simulink library "tip_assist_lib_support"  (Simulink 9.0)
settings: Solver=VariableStepAuto  StartTime=0.0  StopTime=10.0  RelTol=1e-3
undefined symbols (not defined in the file): g, timestep, TipAssistAdvEcmError_t, TipAssistCpmTipOffMode_t, TipAssistLiveWeighStatus_t, TipAssistPayloadType_t, TipAssistSecPfwStatus_t, TipAssistUnsecPfwStatus_t, toa_appNumber, toa_expectedBucketAngNoise, toa_imu_lpf_cutoff_hz, toa_imuBasicOrient, toa_liftBoreDia, toa_liftRodDia, toa_liveLpfCutoffHz, toa_liveSpillRateLpfCutoffHz, toa_mcGroundCombBucketAng, toa_mcGroundCombLiftNormAng, toa_mcGroundLiftNormAng, toa_noSlidingAngle, toa_payload_target_ov_val, toa_payloadTargetMin, toa_pfwLpfCutoffHz, toa_pfwResetLpfCutoffHz, toa_pfwResetStatsBound, toa_pfwResetStatsConf, toa_pfwTiltNormRackThresh, toa_pfwTravelExtentLower, toa_pfwTravelExtentUpper, toa_ratedPayload, toa_reposeMarginAng, toa_sendCpmLiveLpfCutoffHz, toa_sendToCpmMinPrecision, toa_tiltBoreDia, toa_tiltNumCyl, toa_tiltRodDia, toa_toolBcAngle, toa_toolBcLength
libraries: lib_CATutils_Utilities_ApplyName_v2 x113, simulink x18, tip_assist_lib x14, lib_CATutils_Filters_1Pole_LowPass x6, simulink_extras x5, lib_CATutils_Override x3, lib_CATutils_Hysteresis_Latch x3, lib_CATutils_Timer_Countdown x3, tip_assist_lib_support x2
(part 4 of 4)

== matlab function Tip-Off Assist Support Lib/Tip-Off Assist Payload/Pseudo-Frictionless Weigh/Weighing Statistics, Notch, No Latch/Two Sided Confidence Limit ==
  data: confidence input double; bound output double; stdev input double
function bound = TwoSidedConfBound(confidence, stdev)
% Calculates the size of a confidence interval in terms of half its width.
%
% Inputs:
%   confidence
%   Confidence that the resulting bound will enclose the true value.
%
%   stdev
%   The observed standard deviation, expressed in the same units as
%   bound. Can be thought of as defining the scale of the normal
%   distribution that we are assuming represents the data we are sampling.
%
%   Potential units for the arguments are percent of rated payload or
%   payload.
%
% Outputs:
%   bound
%   Bound of the confidence interval, expressed in the same units as stdev.
%   
%   For lower bound, the true value will lie above the mean minus this
%   value.
%   The opposite is true for an upper bound.
%   
% Inspired from pcs_calculate_confidence() in pcs_io.c

% Table of confidence vs two-sided confidence interval bound.
% Units of confidence decimal percent and the ratio of standard
% deviation of a standard normal distribution.
xConfidenceTwoSided = [ 0.0, 0.235822844, 0.382924922, 0.516072694, 0.631879747, 0.728667676, 0.806398927, 0.866385543, 0.910869057, 0.942566872, 0.964271153, 0.978551778, 0.987580668, 0.993066052, 0.997300204, 0.999534742, 1.0 ];
yStdevRatio = [ 0.0, 0.3, 0.5, 0.7, 0.9, 1.1, 1.3, 1.5, 1.7, 1.9, 2.1, 2.3, 2.5, 2.7, 3.0, 3.5, 4.0 ];
stdev_ratio = interp1(xConfidenceTwoSided, yStdevRatio, confidence);
bound = stdev_ratio * stdev;

== matlab function Tip-Off Assist Support Lib/EEF IMU to NEEF gravity vector/EEF vector to NEEF vector ==
  data: eefVector input double; neefVector output double; steeringAngle input double
function neefVector  = fcn(eefVector, steeringAngle)
% Transforms a vector on the EEF to a vector on the NEEF via steering angle
rotAxis = [0; 1; 0];               % Steering right is positive angle
angle = steeringAngle;

% Form rotation matrix
crossProductMatrix = [
    0,          -rotAxis(3),  rotAxis(2);
     rotAxis(3), 0,          -rotAxis(1);
    -rotAxis(2), rotAxis(1),  0
];
tensorProduct = rotAxis * transpose(rotAxis);
rotMatrix = cos(angle) * eye(3) + sin(angle) * crossProductMatrix + ...
    (1 - cos(angle)) * tensorProduct;

neefVector = rotMatrix * eefVector;

== matlab function Tip-Off Assist Support Lib/Tip-Off Assist Payload/Pseudo-Frictionless Weigh/Weighing Statistics, Notch, No Latch/One Sided Confidence Limit ==
  data: confidence input double; bound output double; stdev input double
function bound = oneSidedConfBound(confidence, stdev)
% Calculates the size of a confidence interval in terms of half its width.
%
% Inputs:
%   confidence
%   Confidence that the resulting bound will enclose the true value.
%
%   stdev
%   The observed standard deviation, expressed in the same units as
%   bound. Can be thought of as defining the scale of the normal
%   distribution that we are assuming represents the data we are sampling.
%
%   Potential units for the arguments are percent of rated payload or
%   payload.
%
% Outputs:
%   bound
%   Bound of the confidence interval, expressed in the same units as stdev.
%   
%   For lower bound, the true value will lie above the mean minus this
%   value.
%   The opposite is true for an upper bound.
%   
% Inspired from pcs_calculate_confidence() in pcs_io.c

% Table of confidence vs one-sided confidence interval bound.
% Units of confidence decimal percent and the ratio of standard
% deviation of a standard normal distribution.
xConfidenceOneSided = [0.500000000000000,0.617911422000000,0.691462461000000,0.758036347000000,0.815939873500000,0.864333838000000,0.903199463500000,0.933192771500000,0.955434528500000,0.971283436000000,0.982135576500000,0.989275889000000,0.993790334000000,0.996533026000000,0.998650102000000,0.999767371000000,1];
yStdevRatio = [ 0.0, 0.3, 0.5, 0.7, 0.9, 1.1, 1.3, 1.5, 1.7, 1.9, 2.1, 2.3, 2.5, 2.7, 3.0, 3.5, 4.0 ];
stdev_ratio = interp1(xConfidenceOneSided, yStdevRatio, confidence);
bound = stdev_ratio * stdev;

== matlab function Tip-Off Assist Support Lib/EEF IMU to NEEF gravity vector/euler angles from rot matrix ==
  data: rotations output double; rotMatrix input double
function rotations  = decomp(rotMatrix)
%   Input:  3x3 rotation matrix
%   Output: 1x3 vector of euler angles in degrees
rotations = zeros(1,3);
rotations(1) = atan2(rotMatrix(3,2),rotMatrix(3,3));
rotations(2) = atan2(-rotMatrix(3,1), (sqrt((rotMatrix(3,2)^2)+(rotMatrix(3,3)^2))));
rotations(3) = atan2(rotMatrix(2,1),rotMatrix(1,1));
% convert back to degrees
for i=1:size(rotations,2)
    rotations(i) = 180*rotations(i)/pi;
end
end

== matlab function Tip-Off Assist Support Lib/Tip-Off Assist Payload/Pseudo-Frictionless Weigh/Weighing Statistics, No Notch, No Latch/One Sided Confidence Limit ==
  data: confidence input double; bound output double; stdev input double
function bound = oneSidedConfBound(confidence, stdev)
% Calculates the size of a confidence interval in terms of half its width.
%
% Inputs:
%   confidence
%   Confidence that the resulting bound will enclose the true value.
%
%   stdev
%   The observed standard deviation, expressed in the same units as
%   bound. Can be thought of as defining the scale of the normal
%   distribution that we are assuming represents the data we are sampling.
%
%   Potential units for the arguments are percent of rated payload or
%   payload.
%
% Outputs:
%   bound
%   Bound of the confidence interval, expressed in the same units as stdev.
%   
%   For lower bound, the true value will lie above the mean minus this
%   value.
%   The opposite is true for an upper bound.
%   
% Inspired from pcs_calculate_confidence() in pcs_io.c

% Table of confidence vs one-sided confidence interval bound.
% Units of confidence decimal percent and the ratio of standard
% deviation of a standard normal distribution.
xConfidenceOneSided = [0.500000000000000,0.617911422000000,0.691462461000000,0.758036347000000,0.815939873500000,0.864333838000000,0.903199463500000,0.933192771500000,0.955434528500000,0.971283436000000,0.982135576500000,0.989275889000000,0.993790334000000,0.996533026000000,0.998650102000000,0.999767371000000,1];
yStdevRatio = [ 0.0, 0.3, 0.5, 0.7, 0.9, 1.1, 1.3, 1.5, 1.7, 1.9, 2.1, 2.3, 2.5, 2.7, 3.0, 3.5, 4.0 ];
stdev_ratio = interp1(xConfidenceOneSided, yStdevRatio, confidence);
bound = stdev_ratio * stdev;

== matlab function Tip-Off Assist Support Lib/Tip-Off Assist Payload/Pseudo-Frictionless Weigh/Weighing Statistics, No Notch, No Latch/Two Sided Confidence Limit ==
  data: confidence input double; bound output double; stdev input double
function bound = TwoSidedConfBound(confidence, stdev)
% Calculates the size of a confidence interval in terms of half its width.
%
% Inputs:
%   confidence
%   Confidence that the resulting bound will enclose the true value.
%
%   stdev
%   The observed standard deviation, expressed in the same units as
%   bound. Can be thought of as defining the scale of the normal
%   distribution that we are assuming represents the data we are sampling.
%
%   Potential units for the arguments are percent of rated payload or
%   payload.
%
% Outputs:
%   bound
%   Bound of the confidence interval, expressed in the same units as stdev.
%   
%   For lower bound, the true value will lie above the mean minus this
%   value.
%   The opposite is true for an upper bound.
%   
% Inspired from pcs_calculate_confidence() in pcs_io.c

% Table of confidence vs two-sided confidence interval bound.
% Units of confidence decimal percent and the ratio of standard
% deviation of a standard normal distribution.
xConfidenceTwoSided = [ 0.0, 0.235822844, 0.382924922, 0.516072694, 0.631879747, 0.728667676, 0.806398927, 0.866385543, 0.910869057, 0.942566872, 0.964271153, 0.978551778, 0.987580668, 0.993066052, 0.997300204, 0.999534742, 1.0 ];
yStdevRatio = [ 0.0, 0.3, 0.5, 0.7, 0.9, 1.1, 1.3, 1.5, 1.7, 1.9, 2.1, 2.3, 2.5, 2.7, 3.0, 3.5, 4.0 ];
stdev_ratio = interp1(xConfidenceTwoSided, yStdevRatio, confidence);
bound = stdev_ratio * stdev;

== matlab function Tip-Off Assist Support Lib/EEF IMU to NEEF gravity vector/rotation matrix calc from two vectors ==
  data: level_vec_meas input double; rotMatrix output double; level_vec_act input double; rotAxis output double; angle output double
function [rotMatrix, rotAxis, angle] = fcn(level_vec_meas, level_vec_act)
% Should match output of:
%     vrrotvec2mat(vrrotvec(level_vec_meas, level_vec_act))

if all(level_vec_meas == level_vec_act)
    % No transform necessary, return identity matrix
    rotAxis = single([9999; 9999; 9999]);
    angle = single(9999);
    rotMatrix = single(eye(3));
    return
end
    
a = level_vec_meas;
b = level_vec_act;

cp = cross(a, b);
cpNorm = norm(cp);

rotAxis = cp/cpNorm;
angle_rad = atan(cpNorm/dot(a, b));
angle = angle_rad * 180.0 / pi;

% Form rotation matrix
crossProductMatrix = [
    0,          -rotAxis(3),  rotAxis(2);
     rotAxis(3), 0,          -rotAxis(1);
    -rotAxis(2), rotAxis(1),  0
];
tensorProduct = rotAxis * transpose(rotAxis);
rotMatrix = cos(angle_rad) * eye(3) + sin(angle_rad) * crossProductMatrix + ...
    (1 - cos(angle_rad)) * tensorProduct;

== matlab function Tip-Off Assist Support Lib/Tip-Off Assist Payload/Pseudo-Frictionless Weigh/Variance Anti-Noise Filter1/MATLAB Function ==
  data: u input double; y output double; reset input double
function y = movingAverage(u, reset)

persistent lastSample
if isempty(lastSample) || reset
    lastSample = u;
end
y = (u + lastSample) / 2;
lastSample = u;

== stateflow chart Tip-Off Assist Support Lib/Tip-Off Assist Payload/Pseudo-Frictionless Weigh/Notch filter/NotchFilter/Filter ==
  state Update
    du: updateFilter();
  state initFilter [function]
    (default) -> (junction 133) : {
        | q = (cf*cf*ts*ts)/4.0c;
        | r = cf*ts;
        | p = 1.0c + q;
        | s = 2.0c * (q - 1.0c);
        | t = p + r;
        |
        | alpha = p / t;
        | beta = s / t;
        | gamma = r / t;
        | }
    (junction 133) -> (junction 134) : {
        | rawHist[0] = raw;
        | rawHist[1] = raw;
        | rawHist[2] = raw;
        | }
    (junction 134) -> (junction 135) : {
        | filtHist[0] = raw;
        | filtHist[1] = raw;
        | filtHist[2] = raw;
        | }
    (junction 135) -> (junction 136) : {
        | filtered = filtHist[0];
        | }
  state updateFilter [function]
    (default) -> (junction 141) : {
        | rawHist[2] = rawHist[1];
        | rawHist[1] = rawHist[0];
        | rawHist[0] = raw;
        | }
    (junction 141) -> (junction 142) : {
        | filtHist[2] = filtHist[1];
        | filtHist[1] = filtHist[0];
        | filtHist[0] = (alpha * (rawHist[0] + rawHist[2] - filtHist[2])) + (beta * (rawHist[1] - filtHist[1])) + (gamma * filtHist[2]);
        | }
    (junction 142) -> (junction 143) : {
        | filtered = filtHist[0];
        | }
  (default) -> (junction 157)
  Update -> (junction 157) : [reset]
  (junction 157) -> Update : {initFilter();}
  data: q temporary single; r temporary single; p temporary single; s temporary single; t temporary single; raw input single; reset input boolean; ts input single; cf input single; filtered output single; rawHist local single size=3; filtHist local single size=3; alpha local single; beta local single; gamma local single

== stateflow chart Tip-Off Assist Support Lib/Tip-Off Assist Payload/Pseudo-Frictionless Weigh/Notch filter/NotchFilter1/Filter ==
  state Update
    du: updateFilter();
  state initFilter [function]
    (default) -> (junction 171) : {
        | q = (cf*cf*ts*ts)/4.0c;
        | r = cf*ts;
        | p = 1.0c + q;
        | s = 2.0c * (q - 1.0c);
        | t = p + r;
        |
        | alpha = p / t;
        | beta = s / t;
        | gamma = r / t;
        | }
    (junction 171) -> (junction 172) : {
        | rawHist[0] = raw;
        | rawHist[1] = raw;
        | rawHist[2] = raw;
        | }
    (junction 172) -> (junction 173) : {
        | filtHist[0] = raw;
        | filtHist[1] = raw;
        | filtHist[2] = raw;
        | }
    (junction 173) -> (junction 174) : {
        | filtered = filtHist[0];
        | }
  state updateFilter [function]
    (default) -> (junction 179) : {
        | rawHist[2] = rawHist[1];
        | rawHist[1] = rawHist[0];
        | rawHist[0] = raw;
        | }
    (junction 179) -> (junction 180) : {
        | filtHist[2] = filtHist[1];
        | filtHist[1] = filtHist[0];
        | filtHist[0] = (alpha * (rawHist[0] + rawHist[2] - filtHist[2])) + (beta * (rawHist[1] - filtHist[1])) + (gamma * filtHist[2]);
        | }
    (junction 180) -> (junction 181) : {
        | filtered = filtHist[0];
        | }
  (default) -> (junction 195)
  Update -> (junction 195) : [reset]
  (junction 195) -> Update : {initFilter();}
  data: q temporary single; r temporary single; p temporary single; s temporary single; t temporary single; raw input single; reset input boolean; ts input single; cf input single; filtered output single; rawHist local single size=3; filtHist local single size=3; alpha local single; beta local single; gamma local single

== stateflow chart Tip-Off Assist Support Lib/Tip-Off Assist Payload/Pseudo-Frictionless Weigh/Notch filter/NotchFilter2/Filter ==
  state Update
    du: updateFilter();
  state initFilter [function]
    (default) -> (junction 209) : {
        | q = (cf*cf*ts*ts)/4.0c;
        | r = cf*ts;
        | p = 1.0c + q;
        | s = 2.0c * (q - 1.0c);
        | t = p + r;
        |
        | alpha = p / t;
        | beta = s / t;
        | gamma = r / t;
        | }
    (junction 209) -> (junction 210) : {
        | rawHist[0] = raw;
        | rawHist[1] = raw;
        | rawHist[2] = raw;
        | }
    (junction 210) -> (junction 211) : {
        | filtHist[0] = raw;
        | filtHist[1] = raw;
        | filtHist[2] = raw;
        | }
    (junction 211) -> (junction 212) : {
        | filtered = filtHist[0];
        | }
  state updateFilter [function]
    (default) -> (junction 217) : {
        | rawHist[2] = rawHist[1];
        | rawHist[1] = rawHist[0];
        | rawHist[0] = raw;
        | }
    (junction 217) -> (junction 218) : {
        | filtHist[2] = filtHist[1];
        | filtHist[1] = filtHist[0];
        | filtHist[0] = (alpha * (rawHist[0] + rawHist[2] - filtHist[2])) + (beta * (rawHist[1] - filtHist[1])) + (gamma * filtHist[2]);
        | }
    (junction 218) -> (junction 219) : {
        | filtered = filtHist[0];
        | }
  (default) -> (junction 233)
  Update -> (junction 233) : [reset]
  (junction 233) -> Update : {initFilter();}
  data: q temporary single; r temporary single; p temporary single; s temporary single; t temporary single; raw input single; reset input boolean; ts input single; cf input single; filtered output single; rawHist local single size=3; filtHist local single size=3; alpha local single; beta local single; gamma local single

== matlab function Tip-Off Assist Support Lib/Tip-Off Assist Payload/Pseudo-Frictionless Weigh/Statistics Estimation1/Two Sided St. Dev. from Bound ==
  data: confidence input double; stdev output double; bound input double
function stdev = TwoSidedConfBound(confidence, bound)
% Calculates the st. dev. of a confidence interval in terms of half its width.
%
% Inputs:
%   confidence
%   Confidence that the input bound will enclose the true value.
%
%   bound
%   Bound of the confidence interval, expressed in the same units as stdev.
%   
%   For lower bound, the true value will lie above the mean minus this
%   value.
%   The opposite is true for an upper bound.
%
%   Potential units for the arguments are percent of rated payload or
%   payload.
%
% Outputs:
%   stdev
%   The standard deviation, expressed in the same units as
%   bound, that corresponds to the given bound. Can be thought of as
%   describing the scale of the normal distribution whose confidence
%   interval with given bounds results in the given confidence.
%   
% Inspired from pcs_calculate_confidence() in pcs_io.c

% Table of confidence vs two-sided confidence interval bound.
% Units of confidence decimal percent and the ratio of standard
% deviation of a standard normal distribution.
xConfidenceTwoSided = [ 0.0, 0.235822844, 0.382924922, 0.516072694, 0.631879747, 0.728667676, 0.806398927, 0.866385543, 0.910869057, 0.942566872, 0.964271153, 0.978551778, 0.987580668, 0.993066052, 0.997300204, 0.999534742, 1.0 ];
yStdevRatio = [ 0.0, 0.3, 0.5, 0.7, 0.9, 1.1, 1.3, 1.5, 1.7, 1.9, 2.1, 2.3, 2.5, 2.7, 3.0, 3.5, 4.0 ];
stdev_ratio = interp1(xConfidenceTwoSided, yStdevRatio, confidence);
stdev = bound / stdev_ratio;

== matlab function Tip-Off Assist Support Lib/Tip-Off Assist Payload/Pseudo-Frictionless Weigh/Statistics Estimation2/MATLAB Function ==
  data: newSample input double; meanEst output double; stdevEst output double; filterFactor input double; reset input double; resetSample input double; resetVariance input double
function [meanEst, stdevEst] = fcn(newSample, filterFactor, reset, resetSample, resetVariance)
% Implements a running mean and standard deviation estimate.
% Formula from:
%   Estimation of Variance by a Recursive Equation
%   by M. Melvin Bruce, October 1969, Langley Research Center (NASA)
% Adapted from PCS's pcs_io.c file.

persistent lastMeanEst lastVarianceEst;

% Init to a high variance to ensure confidence is initially low.
% Init to a high mean so the true value is always approached from above,
% which will ensure a non-warmed-up filter errs high, which will cause
% Tip-Off Assist to err low to prevent truck overload.
if isempty(lastMeanEst) || reset
    lastMeanEst = single(resetSample);
    lastVarianceEst = single(resetVariance);
end

A = 1 - filterFactor;   % "A" from the NASA paper
meanEst = A * lastMeanEst + (1.0 - A) * newSample;
varianceEst = A * lastVarianceEst + (1.0 - A) * (1.0 + A) * (newSample - lastMeanEst) * (newSample - lastMeanEst) / 2.0;
stdevEst = sqrt(varianceEst);

% For next time...
lastMeanEst = meanEst;
lastVarianceEst = varianceEst;
end

== matlab function Tip-Off Assist Support Lib/Tip-Off Assist Payload/Pseudo-Frictionless Weigh/Statistics Estimation2/Two Sided St. Dev. from Bound ==
  data: confidence input double; stdev output double; bound input double
function stdev = TwoSidedConfBound(confidence, bound)
% Calculates the st. dev. of a confidence interval in terms of half its width.
%
% Inputs:
%   confidence
%   Confidence that the input bound will enclose the true value.
%
%   bound
%   Bound of the confidence interval, expressed in the same units as stdev.
%   
%   For lower bound, the true value will lie above the mean minus this
%   value.
%   The opposite is true for an upper bound.
%
%   Potential units for the arguments are percent of rated payload or
%   payload.
%
% Outputs:
%   stdev
%   The standard deviation, expressed in the same units as
%   bound, that corresponds to the given bound. Can be thought of as
%   describing the scale of the normal distribution whose confidence
%   interval with given bounds results in the given confidence.
%   
% Inspired from pcs_calculate_confidence() in pcs_io.c

% Table of confidence vs two-sided confidence interval bound.
% Units of confidence decimal percent and the ratio of standard
% deviation of a standard normal distribution.
xConfidenceTwoSided = [ 0.0, 0.235822844, 0.382924922, 0.516072694, 0.631879747, 0.728667676, 0.806398927, 0.866385543, 0.910869057, 0.942566872, 0.964271153, 0.978551778, 0.987580668, 0.993066052, 0.997300204, 0.999534742, 1.0 ];
yStdevRatio = [ 0.0, 0.3, 0.5, 0.7, 0.9, 1.1, 1.3, 1.5, 1.7, 1.9, 2.1, 2.3, 2.5, 2.7, 3.0, 3.5, 4.0 ];
stdev_ratio = interp1(xConfidenceTwoSided, yStdevRatio, confidence);
stdev = bound / stdev_ratio;

== matlab function Tip-Off Assist Support Lib/Tip-Off Assist Payload/Pseudo-Frictionless Weigh/Variance Anti-Noise Filter2/MATLAB Function ==
  data: u input double; y output double; reset input double
function y = movingAverage(u, reset)

persistent lastSample
if isempty(lastSample) || reset
    lastSample = single(u);
end
y = (u + lastSample) / 2;
lastSample = u;

== matlab function Tip-Off Assist Support Lib/Tip-Off Assist Payload/Pseudo-Frictionless Weigh/Unsecure Payload Status ==
  data: inputsBad input double; warm input double; status output double; measCondOk input double
function status = unsecurePfwStatus(inputsBad, warm, measCondOk)

if inputsBad
    status = TipAssistUnsecPfwStatus_t.FAULT;
elseif warm && measCondOk
    % Let consumers know that PFW is valid and may improve in confidence
    status = TipAssistUnsecPfwStatus_t.VALID;
elseif ~warm && measCondOk
    % Let consumers know that PFW is likely about to become valid
    status = TipAssistUnsecPfwStatus_t.PENDING;
else
    status = TipAssistUnsecPfwStatus_t.INVALID;
end

== matlab function Tip-Off Assist Support Lib/Tip-Off Assist Payload/Live Weigh/MATLAB Function1 ==
  data: timestep input double; lowPassFilterFactor output double; lowPassFilterCutoffHz input double
function lowPassFilterFactor = calcFilterFactor(timestep, lowPassFilterCutoffHz)

% Low-pass filter cutoff (rad/s)
cutoff = lowPassFilterCutoffHz * (2 * pi);
% Low-pass filter angle (rad)
angle = cutoff * timestep;
% Filter factor corresponding to cutoff
lowPassFilterFactor = ...
    (cos(angle) - 1) + sqrt((cos(angle) - 3) * (cos(angle) - 1));

== stateflow chart Tip-Off Assist Support Lib/Tip-Off Assist Payload/Live Weigh/Notch filter/NotchFilter/Filter ==
  state Update
    du: updateFilter();
  state initFilter [function]
    (default) -> (junction 300) : {
        | q = (cf*cf*ts*ts)/4.0c;
        | r = cf*ts;
        | p = 1.0c + q;
        | s = 2.0c * (q - 1.0c);
        | t = p + r;
        |
        | alpha = p / t;
        | beta = s / t;
        | gamma = r / t;
        | }
    (junction 300) -> (junction 301) : {
        | rawHist[0] = raw;
        | rawHist[1] = raw;
        | rawHist[2] = raw;
        | }
    (junction 301) -> (junction 302) : {
        | filtHist[0] = raw;
        | filtHist[1] = raw;
        | filtHist[2] = raw;
        | }
    (junction 302) -> (junction 303) : {
        | filtered = filtHist[0];
        | }
  state updateFilter [function]
    (default) -> (junction 308) : {
        | rawHist[2] = rawHist[1];
        | rawHist[1] = rawHist[0];
        | rawHist[0] = raw;
        | }
    (junction 308) -> (junction 309) : {
        | filtHist[2] = filtHist[1];
        | filtHist[1] = filtHist[0];
        | filtHist[0] = (alpha * (rawHist[0] + rawHist[2] - filtHist[2])) + (beta * (rawHist[1] - filtHist[1])) + (gamma * filtHist[2]);
        | }
    (junction 309) -> (junction 310) : {
        | filtered = filtHist[0];
        | }
  (default) -> (junction 324)
  Update -> (junction 324) : [reset]
  (junction 324) -> Update : {initFilter();}
  data: q temporary single; r temporary single; p temporary single; s temporary single; t temporary single; raw input single; reset input boolean; ts input single; cf input single; filtered output single; rawHist local single size=3; filtHist local single size=3; alpha local single; beta local single; gamma local single

== stateflow chart Tip-Off Assist Support Lib/Tip-Off Assist Payload/Live Weigh/Notch filter/NotchFilter1/Filter ==
  state Update
    du: updateFilter();
  state initFilter [function]
    (default) -> (junction 338) : {
        | q = (cf*cf*ts*ts)/4.0c;
        | r = cf*ts;
        | p = 1.0c + q;
        | s = 2.0c * (q - 1.0c);
        | t = p + r;
        |
        | alpha = p / t;
        | beta = s / t;
        | gamma = r / t;
        | }
    (junction 338) -> (junction 339) : {
        | rawHist[0] = raw;
        | rawHist[1] = raw;
        | rawHist[2] = raw;
        | }
    (junction 339) -> (junction 340) : {
        | filtHist[0] = raw;
        | filtHist[1] = raw;
        | filtHist[2] = raw;
        | }
    (junction 340) -> (junction 341) : {
        | filtered = filtHist[0];
        | }
  state updateFilter [function]
    (default) -> (junction 346) : {
        | rawHist[2] = rawHist[1];
        | rawHist[1] = rawHist[0];
        | rawHist[0] = raw;
        | }
    (junction 346) -> (junction 347) : {
        | filtHist[2] = filtHist[1];
        | filtHist[1] = filtHist[0];
        | filtHist[0] = (alpha * (rawHist[0] + rawHist[2] - filtHist[2])) + (beta * (rawHist[1] - filtHist[1])) + (gamma * filtHist[2]);
        | }
    (junction 347) -> (junction 348) : {
        | filtered = filtHist[0];
        | }
  (default) -> (junction 362)
  Update -> (junction 362) : [reset]
  (junction 362) -> Update : {initFilter();}
  data: q temporary single; r temporary single; p temporary single; s temporary single; t temporary single; raw input single; reset input boolean; ts input single; cf input single; filtered output single; rawHist local single size=3; filtHist local single size=3; alpha local single; beta local single; gamma local single

== stateflow chart Tip-Off Assist Support Lib/Tip-Off Assist Payload/Live Weigh/Notch filter/NotchFilter2/Filter ==
  state Update
    du: updateFilter();
  state initFilter [function]
    (default) -> (junction 376) : {
        | q = (cf*cf*ts*ts)/4.0c;
        | r = cf*ts;
        | p = 1.0c + q;
        | s = 2.0c * (q - 1.0c);
        | t = p + r;
        |
        | alpha = p / t;
        | beta = s / t;
        | gamma = r / t;
        | }
    (junction 376) -> (junction 377) : {
        | rawHist[0] = raw;
        | rawHist[1] = raw;
        | rawHist[2] = raw;
        | }
    (junction 377) -> (junction 378) : {
        | filtHist[0] = raw;
        | filtHist[1] = raw;
        | filtHist[2] = raw;
        | }
    (junction 378) -> (junction 379) : {
        | filtered = filtHist[0];
        | }
  state updateFilter [function]
    (default) -> (junction 384) : {
        | rawHist[2] = rawHist[1];
        | rawHist[1] = rawHist[0];
        | rawHist[0] = raw;
        | }
    (junction 384) -> (junction 385) : {
        | filtHist[2] = filtHist[1];
        | filtHist[1] = filtHist[0];
        | filtHist[0] = (alpha * (rawHist[0] + rawHist[2] - filtHist[2])) + (beta * (rawHist[1] - filtHist[1])) + (gamma * filtHist[2]);
        | }
    (junction 385) -> (junction 386) : {
        | filtered = filtHist[0];
        | }
  (default) -> (junction 400)
  Update -> (junction 400) : [reset]
  (junction 400) -> Update : {initFilter();}
  data: q temporary single; r temporary single; p temporary single; s temporary single; t temporary single; raw input single; reset input boolean; ts input single; cf input single; filtered output single; rawHist local single size=3; filtHist local single size=3; alpha local single; beta local single; gamma local single

== matlab function Tip-Off Assist Support Lib/Tip-Off Assist Payload/Pseudo-Frictionless Weigh/MATLAB Function1 ==
  data: timestep input double; lowPassFilterFactor output double; lowPassFilterCutoffHz input double
function lowPassFilterFactor = calcFilterFactor(timestep, lowPassFilterCutoffHz)

% Low-pass filter cutoff (rad/s)
cutoff = lowPassFilterCutoffHz * (2 * pi);
% Low-pass filter angle (rad)
angle = cutoff * timestep;
% Filter factor corresponding to cutoff
lowPassFilterFactor = ...
    (cos(angle) - 1) + sqrt((cos(angle) - 3) * (cos(angle) - 1));

== matlab function Tip-Off Assist Support Lib/Lift Friction Compensation/MATLAB Function ==
  data: rawPress input double; liftCmd input double; compPress output double; fricCoeff input double; fricOffset input double
function compPress = fcn(rawPress, liftCmd, fricCoeff, fricOffset)
% rawPress
%   Equivalent HE pressure in kPa
% liftCmd
%   Lift command with
% fricCoeff
%   Friction coefficient in units of kPa of friction / raw kPa
% fricOffset
%   Friction offset in units of kPa

if liftCmd < 0.0        % Lower
    compPress = (1 + fricCoeff) * rawPress + fricOffset;
elseif liftCmd == 0.0   % Hold
    compPress = rawPress;
elseif liftCmd > 0.0    % Raise
    compPress = (1 - fricCoeff) * rawPress - fricOffset;
else
    % Unexpected, so propogate value that triggers bad status
    compPress = single(NaN);
end
